simulink model "vrm_plus_ff_return_backup"  (R2013a)
settings: Solver=ode4  SolverMode=SingleTasking  StartTime=0.0  StopTime=inf  FixedStep=0.0005  RelTol=1e-3
StartFcn:
  |  warndlg('Dexterit-E models cannot run under simulation. Please compile your model and run it from within Dexterit-E.');set_param(bdroot,'SimulationCommand','stop')
model workspace (MAT data in the model file):
  BKIN_STEP_TIME = 0.0005
  col_x = 1
  col_y = 2
  E_TARGET_ON = 3
  E_HOLD_AT_TARGET = 5
  LOGICAL_RADIUS = 4
  START_TARGET_COL = 1
  END_TARGET_COL = 2
  ROTATION_CENTER = 3
  WAIT_AT_1stTARGET_COL = 4
  MAXREACHTIME_COL = 5
  WAIT_AT_2ndTARGET_COL = 6
  ROTATION_TYPE = 8
  ROTATION = 9
  DELAY_POSTTRIAL_COL = 7
  E_STAY_CENTER = 2
  VISUAL_RADIUS = 3
  COLOR = 5
  ALTCOLOR = 6
  A_VISC = 1
  B_VISC = 2
  C_VISC = 3
  D_VISC = 4
  LOAD = 10
  TRAJ_DURATION_COL = 11
undefined symbols (not defined in the file or in its folder): slselsubs
libraries: General x3, KINARM_EP_loads x3, Video x3, KINARM_general x1, simulink x1, KINARM_loads x1
(part 2 of 2)

== matlab function vrm_plus_ff_return_backup/KINARM_HandFeedbackInTarget/Embedded MATLAB InsideTarget ==
  settings: fimath=|
      | fimath(...
      | 'RoundMode', 'floor',...
      | 'OverflowMode', 'wrap',...
      | 'ProductMode', 'KeepLSB', 'ProductWordLength', 32,...
      | 'SumMode', 'KeepLSB', 'SumWordLength', 32,...
      | 'CastBeforeSum', false)
  data: handpos input size=2; target_type input; attribcol input; num_targets input; intarget output; Target_Table input
function intarget = FIsInsideTarget(handpos, target_type, attribcol, num_targets, Target_Table)
% all dimensions in m, rad
% arguments:
% handpos: x,y positions of center of target
% attribcol: columns in target table specifying target attributes.  
% Specific to Target_Type
%	circle:
%	[X0,Y0,r...,rn] where:
%	X0,Y0 : centre of circle
%	r : logical radius of circle (i.e. radius used to determine 'in' or 'out' of target)
%	rn: logical radius of other targets (e.g. 2nd, 3rd) also specified in target row.
%   Up to 4 targets can be specified in a row
% ellipse:
%	[X0,Y0,a,b,t...,an, bn, tn] where:
%	X0,Y0 : centre of ellipse
%	a,b : major, minor radii of ellipse
%	t : rotation of ellipse in degrees
%	an,bn : major, minor radii of ellipse of other targets (e.g. 2nd, 3rd) also specified in target row
%	tn : rotation of ellipse in degrees of other targets (e.g. 2nd, 3rd) also specified in target row
%   Up to 4 targets can be specified in a row


target_col_x=1;
target_col_y=2;

x=handpos(1);
y=handpos(2);

intarget = zeros(size(Target_Table,1),4);

X0 = Target_Table(:,target_col_x)*0.01;			%Target Table sizes in cm in v1.4
Y0 = Target_Table(:,target_col_y)*0.01;			%Target Table sizes in cm in v1.4

deltax=x-X0;
deltay=y-Y0;

INT_MAX=2^32-1;

if target_type==1			%circle
	for target=1:num_targets
		r = Target_Table(:,attribcol(target))*0.01;			%Target Table sizes in cm in v1.4
		% simple euclidean distance
		distance2 = deltax.^2 + deltay.^2;					%distance2 is the square of the distance
	    intarget(:,target) = (distance2 <= r.^2);
	end
elseif target_type==2		%ellipse
	for target=1:num_targets
	    a = Target_Table(:,attribcol(target*3-2))*0.01;			%Target Table sizes in cm in v1.4
	    b = Target_Table(:,attribcol(target*3-1))*0.01;			%Target Table sizes in cm in v1.4	
	    t = Target_Table(:,attribcol(target*3))*(pi / 180.0);	%Target Table angles in degrees in v1.4
		sint=sin(t);
		cost=cos(t);
		xrotate=deltax.*cost+deltay.*sint;		%location of x point in ellipse's coordinate frame
		yrotate=-deltax.*sint+deltay.*cost;		%location of y point in ellipse's coordinate frame
		m=yrotate./xrotate;						%slope of line between the (x,y) to (x0,y0) in ellipse's coordinate frame
		y2sq=1./(1./(m.*a).^2+1./b.^2);			%y2sq is y2^2, where y2 is the intersection of the ellipse and the (x,y) to (x0,y0) line
	    intarget(:,target) = (yrotate.^2 <= y2sq);
    end
elseif target_type==3       %rectangle
    for target=1:num_targets
        w = Target_Table(:,attribcol(target*3-2))*0.01;  %width (sizes in cm in v1.4)
        h = Target_Table(:,attribcol(target*3-1))*0.01;  %height (sizes in cm in v1.4)
        
        if attribcol(target*3) > 0
            t = Target_Table(:,attribcol(target*3))*(pi / 180.0);  %angle (angles in degrees in v1.4)
        else
            t = zeros(size(Target_Table, 1), 1);
        end

        sint=sin(t);
        cost=cos(t);

        xrotate=deltax.*cost + deltay.*sint;   %location of x point in rectangle's coordinate frame
        yrotate=-deltax.*sint + deltay.*cost;  %location of y point in rectangle's coordinate frame

        intarget(:,target) = abs(xrotate) <= w/2 & abs(yrotate) <= h/2;
    end
elseif target_type==4       %line
    for target=1:num_targets
        % treat the line like a rectangle of height h and width w
        % determine height (stroke width) in the same fashion as in Show_Target
        if attribcol(target*3-2) == 0                     %0 column index means stroke width of 0
            h = zeros(size(Target_Table, 1), 1);
        elseif attribcol(target*3-2) < 0                  %-ve column index means stroke width of 1mm
            h = ones(size(Target_Table, 1), 1) .* 0.001;
        else
            h = Target_Table(:,attribcol(target*3-2)) * 0.01;  %target table contains width in cm
        end
        
        ex = Target_Table(:,attribcol(target*3-1))*0.01;  %endpoint in x relative to start point (cm)
        ey = Target_Table(:,attribcol(target*3))*0.01;    %endpoint in y relative to start point (cm)
        
        w = sqrt(ex.^2 + ey.^2);                          %width (cm)
        
        % determine the vector from the line's midpoint to the hand position
        handx = deltax - ex/2;
        handy = deltay - ey/2;
        
        t = atan2(ey, ex);                                %calculate angle of the line (rads)
        sint = sin(t);
        cost = cos(t);
        
        xrotate = handx.*cost + handy.*sint;   %location of x point in rectangle's coordinate frame
        yrotate = -handx.*sint + handy.*cost;  %location of y point in rectangle's coordinate frame
 
        intarget(:,target) = abs(xrotate) <= w/2 & abs(yrotate) <= h/2;
    end
elseif target_type==5  % triangle
    for target=1:num_targets
        w = Target_Table(:,attribcol(target*4-3))*0.01;         %length (sizes in cm in v1.4)
        
        % If a height column of 0 is specified, make the triangle equilateral. Otherwise, use the
        % values for height and peak offset from the target table.
        if attribcol(target*4-2) > 0
            h = Target_Table(:,attribcol(target*4-2))*0.01;  %height (sizes in cm in v1.4)
            p = Target_Table(:,attribcol(target*4-1))*0.01;  %peak offset (sizes in cm in v1.4)
        else
            h = w.*sin(pi/3.0);
            p = zeros(size(Target_Table, 1), 1);
        end
        
        if attribcol(target*4) > 0
            t = Target_Table(:,attribcol(target*4))*(pi / 180.0);  %angle (angles in degrees in v1.4)
        else
            t = zeros(size(Target_Table, 1), 1);
        end
        
        sint = sin(t);
        cost = cos(t);
        
        xrotate = deltax.*cost + deltay.*sint;   %location of x point in triangle's coordinate frame
        yrotate = -deltax.*sint + deltay.*cost;  %location of y point in triangle's coordinate frame
        
        % Begin to find centroid of triangle relative to the point on the base beneath the peak. "Left vertex" 
        % refers to the vertex at the left end of the base, and "right vertex" to the vertex at the right end.
        n = w./2.0 + p;  % distance along base from left vertex to peak
        m = w./2.0 - p;  % distance along base from peak to right vertex

        alpha = atan2(h, n);  % angle between base and line from left vertex to peak
        beta = atan2(h, m);   % angle between base and line from right vertex to peak
        
        length1 = sqrt(h.*h + n.*n) ./ 2.0;  % half length of line from left vertex to peak
        length2 = sqrt(h.*h + m.*m) ./ 2.0;  % half length of line from right vertex to peak

        % Determine slope of line from left vertex to midpoint of line from right vertex to peak.
        slope1 = ones(size(Target_Table, 1), 1) .* INT_MAX;
        
        for i=1:size(Target_Table, 1)
            if abs(w(i) - length2(i)*cos(beta(i))) > 0.0
                slope1(i) = length2(i)*sin(beta(i)) / (w(i) - length2(i)*cos(beta(i)));
            end
        end

        % Determine slope of line from right vertex to midpoint of line from left vertex to peak.
        slope2 = ones(size(Target_Table, 1), 1) .* INT_MAX;

        for i=1:size(Target_Table, 1)
            if abs(w(i) - length1(i)*cos(alpha(i))) > 0.0
                slope2(i) = -length1(i)*sin(alpha(i)) / (w(i) - length1(i)*cos(alpha(i)));
            end
        end

        % Calculate centroid position.
        centroid_x = -(m.*slope2 + n.*slope1) ./ (slope1 - slope2);
        centroid_y = slope1.*(centroid_x + n);

        % Test if the point is under the left side of the peak.
        is_under_left = false(size(Target_Table, 1), 1);

        for i=1:size(Target_Table, 1)
            if n(i) >= 0
                is_under_left(i) = (h(i) + (h(i)/n(i)) * (xrotate(i) + centroid_x(i))) >= (yrotate(i) + centroid_y(i));
            else
                is_under_left(i) = (h(i) + (h(i)/n(i)) * (xrotate(i) + centroid_x(i))) <= (yrotate(i) + centroid_y(i));
            end
        end
        
        % Test if the point is under the right side of the peak.
        is_under_right = false(size(Target_Table, 1), 1);

        for i=1:size(Target_Table, 1)
            if m(i) >= 0
                is_under_right(i) = (h(i) - (h(i)/m(i)) * (xrotate(i) + centroid_x(i))) >= (yrotate(i) + centroid_y(i));
            else
                is_under_right(i) = (h(i) - (h(i)/m(i)) * (xrotate(i) + centroid_x(i))) <= (yrotate(i) + centroid_y(i));
            end
        end
        
        intarget(:,target) = is_under_right & ...            %under right side of peak
                             is_under_left & ...             %under left side of peak
                             (yrotate + centroid_y) >= 0.0;  %above base
    end
end

== matlab function vrm_plus_ff_return_backup/KINARM_HandFeedbackInTarget/Embedded MATLAB WhichHand ==
  settings: fimath=|
      | fimath(...
      | 'RoundMode', 'floor',...
      | 'OverflowMode', 'wrap',...
      | 'ProductMode', 'KeepLSB', 'ProductWordLength', 32,...
      | 'SumMode', 'KeepLSB', 'SumWordLength', 32,...
      | 'CastBeforeSum', false)
  data: use_dominant_hand input; dominant_hand input; hand output; cursor output
function [hand, cursor] = WhichHand(use_dominant_hand, dominant_hand)

if use_dominant_hand==1				%use the dominant hand
	hand=dominant_hand;		
	cursor = 1;
else
	hand=3-dominant_hand;			%use the non-dominant hand. i.e. if dominant_hand=2, hand=1 and vice-versa
	cursor = 2;
end

== matlab function vrm_plus_ff_return_backup/Select_load_mode/Trajectory subsystem/Create_Trajectory/Virtual_Trajectory/Extract_Position ==
  settings: fimath=|
      | fimath(...
      | 'RoundMode', 'floor',...
      | 'OverflowMode', 'wrap',...
      | 'ProductMode', 'KeepLSB', 'ProductWordLength', 32,...
      | 'SumMode', 'KeepLSB', 'SumWordLength', 32,...
      | 'CastBeforeSum', false)
  data: u input; position output
function position = fcn(u)

position=[0,0];	%initialization
if length(u)==2	%input is assumed to be (x,y) position, global coordinates, (m)		
	position=u;
else			%input is assumed to be a VCODE
	position(1)=u(3);
	position(2)=u(4);
end

== matlab function vrm_plus_ff_return_backup/Select_load_mode/Trajectory subsystem/Create_Trajectory/Virtual_Trajectory/Extract_Position1 ==
  settings: fimath=|
      | fimath(...
      | 'RoundMode', 'floor',...
      | 'OverflowMode', 'wrap',...
      | 'ProductMode', 'KeepLSB', 'ProductWordLength', 32,...
      | 'SumMode', 'KeepLSB', 'SumWordLength', 32,...
      | 'CastBeforeSum', false)
  data: u input; position output
function position = fcn(u)

position=[0,0];	%initialization
if length(u)==2	%input is assumed to be (x,y) position, global coordinates, (m)		
	position=u;
else			%input is assumed to be a VCODE
	position(1)=u(3);
	position(2)=u(4);
end

== stateflow chart vrm_plus_ff_return_backup/Select_load_mode/Trajectory subsystem/Create_Trajectory/Virtual_Trajectory/VirtualTrajectory ==
  state Initialization/
    virt_pos = reset_pos;
    // this initialization ensures that the virtual position
    // starts off as something reasonable
    traj_status = 0;   // initialize trajectory status
  state main/
    state wait_for_trigger/
      reset_controller = 0;
    state wait_1_ms_b/
      // wait for controller
      // to be reset
    state on_ramp/
      entry: tick = 0;    // initialize the tick counter
      reset_controller = 0;
      final_pos = target_pos;   // set the final position of the trajectory
      start_pos = virt_pos;   // set the start position of the trajectory
      duration = input_duration;   // store the duration of the trajectory
      traj_status = 1;   // indicate an ongoing trajectory
      during:
      on e_clk: tick++;
      // the trajectory velocity will have a bell shaped profile
      trajectory_shape = tick/duration-sin(2*pi*tick/duration)/(2*pi);
      virt_pos[1] = start_pos[1] + (final_pos[1] - start_pos[1]) * trajectory_shape;
      virt_pos[2] = start_pos[2] + (final_pos[2] - start_pos[2]) * trajectory_shape;
    main -> wait_1_ms_b [order 1] : [(robot_enabled == 1) && (traj_status == -1)]/
        | traj_status = 1;
        | virt_pos = reset_pos;
        | reset_controller = 1;
        | // trajectory was halted and
        | //is now being re-started
    wait_for_trigger -> (junction 20) : e_start
    (junction 20) -> wait_for_trigger [order 2]
    wait_1_ms_b -> (junction 20) : after(1, e_clk)
    (junction 20) -> on_ramp [order 1] : [input_duration>0]
    on_ramp -> wait_for_trigger [order 2] : [robot_enabled == 0]/
        | traj_status = -1;
        | // robot disabled
    on_ramp -> wait_for_trigger [order 1] : after(duration, e_clk)/
        | traj_status = 0
        | // trajectory completed
  state wait_1_ms/
    // wait for controller
    // to be reset
  state task_not_running/
    // wait for task_status to change
    // keep updating virt_pos so that the feedback
    // controller output, which is filtered, does not become
    // huge, resulting in a 'bump' if we don't do this.
    traj_status = 0;
    reset_controller = 0;
    during:
    virt_pos = reset_pos;
  (default) -> Initialization
  Initialization -> wait_for_trigger
  wait_1_ms -> wait_for_trigger : after(1, e_clk)
  task_not_running -> wait_1_ms : [task_status > 0]/
      | reset_controller = 1;
      | // task is running again,
      | // so reset position controller
  main -> task_not_running [order 1] : [task_status == 0]/
      | // means that run_status == 0
      | // AND that torque scaling at
      | // end of task is finished
  data: input_duration input double; target_pos input double size=[1 2]; tick local double; duration local double; reset_pos input double size=[1 2]; task_status input double; pi constant double =3.14159265358979; trajectory_shape local double; virt_pos output double size=[1 2]; traj_status output double; robot_enabled input double; start_pos local double size=[1 2]; final_pos local double size=[1 2]; reset_controller output double
  events: e_clk input RISING_EDGE_EVENT; e_start input RISING_EDGE_EVENT

== matlab function vrm_plus_ff_return_backup/Select_load_mode/Trajectory subsystem/Create_Trajectory/get_arm_info ==
  settings: fimath=|
      | fimath(...
      | 'RoundMode', 'floor',...
      | 'OverflowMode', 'wrap',...
      | 'ProductMode', 'KeepLSB', 'ProductWordLength', 32,...
      | 'SumMode', 'KeepLSB', 'SumWordLength', 32,...
      | 'CastBeforeSum', false)
  data: position output; task_status output; use_dom_hand input; kinarm_data input; run_status input; scaling input; robot_enabled output
function [position, task_status, robot_enabled]  = fcn(use_dom_hand, kinarm_data, run_status, scaling)
%
% get current hand position and robot enabled status
%
% May 2009
%

hpx_index = 23;
hpy_index = 24;
robot_disabled_index = 37;

%determine which arm to apply the load to
dominant_hand=kinarm_data(3,1);						%kinarm_data(3,1) tells which arm is the dominant arm
if use_dom_hand == 1
	feedback_arm = dominant_hand;
else
	feedback_arm = 3 - dominant_hand;
end

hpx = kinarm_data( feedback_arm, hpx_index );
hpy = kinarm_data( feedback_arm, hpy_index );
position = [hpx hpy];

if kinarm_data( feedback_arm, robot_disabled_index ) == 0;
    robot_enabled = 1;
else
    robot_enabled = 0;
end

% if the task has stopped/paused (i.e. run_status == 0) AND the torques outputs
% have scaled down to 0, then set the task_status = 0.
if run_status == 0 && scaling(feedback_arm) == 0
    task_status = 0;
else
    task_status = 1;
end

== matlab function vrm_plus_ff_return_backup/Select_load_mode/Trajectory subsystem/calculate robot scaling/MATLAB Function ==
  data: robot_type input; scaling output; exo_scaling input; ep_scaling input
function scaling = fcn(robot_type, exo_scaling, ep_scaling)
%#codegen

scaling = [0, 0];

%0 = EXO, 1 = EP, 2 = NHP
for n=1:2
    if robot_type(n) == 1
        scaling(n) = ep_scaling(n);
    else
        scaling(n) = exo_scaling(n);
    end
end
